simulink model "vdynblksskidpad_final"  (R2026b)
settings: Solver=ode23t  StopTime=inf  RelTol=5e-3
model workspace (MAT data in the model file):
  Eng : object (value not decoded)
  Nmtr = 11.5
  StartupTrim : object (value not decoded)
  SteerLim = 60
  TrackPoints = [-15 -12 -9 -6 -3 5.58745102111e-16 2.81978007367 5.36354042717 7.38228007367 8.67839071119 9.125 8.67839071119 ... (270 elements, 90x3)]
  Trans : object (value not decoded)
  Ts = 0.02
  VEH : object (value not decoded)
values from neighbouring files (symbols this model uses):
  n = size(e.Data,2)    [plot_skidpad_signals.m]
  z = tsMatrix(out.diagWheel.z)    [skidpad_settle_start.m]
symbols that are objects in the model workspace (value not decoded): Eng, StartupTrim, Trans, VEH
undefined symbols (not defined in the file or in its folder): BdyFrm, InertFrm, magnitude
libraries: autolibsharedcoupling x11, simulink x8, sim3dlib x7, autolibshareddiff x5, autolibutils x4, sim3dautolib x3, vehdynlibtirecommon x3, sharedtransform x3, vehdynlibdriver x2, vehdynlibsteering x2, vehdynlibeom x2, vehdynlibviscommon x2
(part 3 of 5)

== system vdynblksskidpad_final/Formula Student Vehicle/Simulink Physics - 7DOF/Powertrain & Driveline/Final Drive/All Wheel Drive ==
  DrvShfTrq : Inport
  Omega : Inport  Port=2
  Demux1 : Demux  Outputs=2
  Demux2 : Demux  Outputs=2
  Demux3 : Demux  Outputs=2
  Limited Slip Differential : autolibshareddiff/Limited Slip Differential  DiffEffModelPopup=Constant  InterpMethod=Linear point-slope  extTamb=off  shaftSwitchMask=To the left of center-line  Ndiff=4  Jd=.1  bd=1e-3  Jw1=.1  bw1=1e-3  Jw2=.1  bw2=1e-3  omegaw1o=0  omegaw2o=0  eta=1  eta_tbl=reshape([0.64 0.76 0.8 0.81 0.83 0.84 0.84 0.56 0.73 0.78 0.8 0.83 0.84 0.84 0.54 0.71 0.77 0.8 0.82 0.84 0.84 0.53 0.71 0.77 0.8 0.83 0.84 0.84 0.51 0.71 0.77 0.8 0.83 0.84 0.85 0.52 0.7 0.77 0.8 0.83 0.84 0.85 0.51 0.71 0.76 0.79 0.83 0.84 0.85 0.5 0.69 0.76 0.79 0.82 0.84 0.85 0.45 0.68 0.75 0.78 0.82 0.84 0.85 0.43 0.67 0.74 0.78 0.81 0.83 0.84 0.38 0.63 0.71 0.75 0.8 0.82 0.83 0.81 0.86 0.88 0.89 0.89 0.89 0.9 0.77 0.85 0.87 0.88 0.89 0.9 0.9 0.72 0.82 0.86 0.87 0.88 0.89 0.9 0.68 0.8 0.84 0.86 0.88 0.89 0.89 0.67 0.8 0.84 0.86 0.88 0.89 0.9 0.67 0.8 0.84 0.86 0.88 0.89 0.9 0.65 0.8 0.84 0.86 0.88 0.89 0.9 0.64 0.79 0.83 0.86 0.88 0.89 0.9 0.63 0.78 0.83 0.86 0.88 0.89 0.9 0.59 0.76 0.82 0.85 0.87 0.89 0.9 0.53 0.73 0.8 0.83 0.86 0.88 0.89], 7, 11, 2)  Trq_bpts=[25, 50, 75, 100, 150, 200, 250]  omega_bpts=[52.4 78.5 105 131 157 183 209 262 314 419 524]  Temp_bpts=[290 358]  Tamb=297.15  couplingType=Pre-loaded ideal clutch  Ndisks=4  Reff=.20  Fc=500  muc=[.16 0.13 0.115 0.11 0.105 0.1025 0.10125]  dw=[0 10 20 40 60 80 100]  Tdw=[-100, -90, -50, -5, 0, 5, 50, 90, 100]  dwT=[-200, -175, -100, - 50, 0, 50, 100, 175, 200]  TTin=[-200 -175 -100 - 50 0 50 100 175 200]  Tin=[-200 -175 -100 - 50 0 50 100 175 200]  tauC=.01  IdealInterpMethod=Linear point-slope  IdealExtrapMethod=Clip  TdwInterpMethod=Linear point-slope  TdwExtrapMethod=Clip  TTinInterpMethod=Linear point-slope  TTinExtrapMethod=Clip  maxAbsSpd=5e3  aMode=2
      settings: LibrarySourceBlock=vdynlib/Powertrain/Drivetrain/Final Drive Unit/Limited Slip Differential
  Open Differential : autolibshareddiff/Open Differential  DiffEffModelPopup=Constant  InterpMethod=Linear point-slope  extTamb=off  shaftSwitchMask=To the left of center-line  Ndiff=4  Jd=.1  bd=1e-3  Jw1=.1  bw1=1e-3  Jw2=.1  bw2=1e-3  omegaw1o=0  omegaw2o=0  eta=1  eta_tbl=reshape([0.64 0.76 0.8 0.81 0.83 0.84 0.84 0.56 0.73 0.78 0.8 0.83 0.84 0.84 0.54 0.71 0.77 0.8 0.82 0.84 0.84 0.53 0.71 0.77 0.8 0.83 0.84 0.84 0.51 0.71 0.77 0.8 0.83 0.84 0.85 0.52 0.7 0.77 0.8 0.83 0.84 0.85 0.51 0.71 0.76 0.79 0.83 0.84 0.85 0.5 0.69 0.76 0.79 0.82 0.84 0.85 0.45 0.68 0.75 0.78 0.82 0.84 0.85 0.43 0.67 0.74 0.78 0.81 0.83 0.84 0.38 0.63 0.71 0.75 0.8 0.82 0.83 0.81 0.86 0.88 0.89 0.89 0.89 0.9 0.77 0.85 0.87 0.88 0.89 0.9 0.9 0.72 0.82 0.86 0.87 0.88 0.89 0.9 0.68 0.8 0.84 0.86 0.88 0.89 0.89 0.67 0.8 0.84 0.86 0.88 0.89 0.9 0.67 0.8 0.84 0.86 0.88 0.89 0.9 0.65 0.8 0.84 0.86 0.88 0.89 0.9 0.64 0.79 0.83 0.86 0.88 0.89 0.9 0.63 0.78 0.83 0.86 0.88 0.89 0.9 0.59 0.76 0.82 0.85 0.87 0.89 0.9 0.53 0.73 0.8 0.83 0.86 0.88 0.89], 7, 11, 2)  Trq_bpts=[25, 50, 75, 100, 150, 200, 250]  omega_bpts=[52.4 78.5 105 131 157 183 209 262 314 419 524]  Temp_bpts=[290 358]  Tamb=297.15  maxAbsSpd=5e3  aMode=2
      settings: LibrarySourceBlock=vdynlib/Powertrain/Drivetrain/Final Drive Unit/Open Differential
  Terminator : Terminator
  Terminator1 : Terminator
  Terminator2 : Terminator
  Torsional Compliance{,1..3} (4 alike) : autolibsharedcoupling/Torsional Compliance  port_config=Simulink  extInfo=off  k=5e3  b=50  theta_o=0  domega_o=0  omega_c=150  blkID=0  aMode=2
      settings: LibrarySourceBlock=vdynlib/Powertrain/Drivetrain/Couplings/Torsional Compliance
  Torsional Compliance4 : autolibsharedcoupling/Torsional Compliance  port_config=Simulink  extInfo=off  k=1e4  b=1e2  theta_o=0  domega_o=0  omega_c=3000  blkID=0  aMode=2
      settings: LibrarySourceBlock=vdynlib/Powertrain/Drivetrain/Couplings/Torsional Compliance
  Torsional Compliance5 : autolibsharedcoupling/Torsional Compliance  port_config=Simulink  extInfo=off  k=1e4  b=1e2  theta_o=0  domega_o=0  omega_c=3000  blkID=0  aMode=2
      settings: LibrarySourceBlock=vdynlib/Powertrain/Drivetrain/Couplings/Torsional Compliance
  Transfer Case : autolibshareddiff/Transfer Case  DiffEffModelPopup=Constant  InterpMethod=Linear point-slope  extTamb=off  TrqSplitRatioMode=off  SpdLockMode=off  shaftSwitchMask=To the left of center-line  Ndiff=1  Jd=.1  bd=1e-3  Jw1=.1  bw1=1e-3  Jw2=.1  bw2=1e-3  omegaw1o=0  omegaw2o=0  eta=1  eta_tbl=reshape([0.64 0.76 0.8 0.81 0.83 0.84 0.84 0.56 0.73 0.78 0.8 0.83 0.84 0.84 0.54 0.71 0.77 0.8 0.82 0.84 0.84 0.53 0.71 0.77 0.8 0.83 0.84 0.84 0.51 0.71 0.77 0.8 0.83 0.84 0.85 0.52 0.7 0.77 0.8 0.83 0.84 0.85 0.51 0.71 0.76 0.79 0.83 0.84 0.85 0.5 0.69 0.76 0.79 0.82 0.84 0.85 0.45 0.68 0.75 0.78 0.82 0.84 0.85 0.43 0.67 0.74 0.78 0.81 0.83 0.84 0.38 0.63 0.71 0.75 0.8 0.82 0.83 0.81 0.86 0.88 0.89 0.89 0.89 0.9 0.77 0.85 0.87 0.88 0.89 0.9 0.9 0.72 0.82 0.86 0.87 0.88 0.89 0.9 0.68 0.8 0.84 0.86 0.88 0.89 0.89 0.67 0.8 0.84 0.86 0.88 0.89 0.9 0.67 0.8 0.84 0.86 0.88 0.89 0.9 0.65 0.8 0.84 0.86 0.88 0.89 0.9 0.64 0.79 0.83 0.86 0.88 0.89 0.9 0.63 0.78 0.83 0.86 0.88 0.89 0.9 0.59 0.76 0.82 0.85 0.87 0.89 0.9 0.53 0.73 0.8 0.83 0.86 0.88 0.89], 7, 11, 2)  Trq_bpts=[25, 50, 75, 100, 150, 200, 250]  omega_bpts=[52.4 78.5 105 131 157 183 209 262 314 419 524]  Temp_bpts=[290 358]  Tamb=297.15  maxAbsSpd=5e3  aMode=2  TrqSplitRatio=0.5  SpdLock=0
      settings: LibrarySourceBlock=vdynlib/Powertrain/Drivetrain/Final Drive Unit/Transfer Case
  Vector Concatenate : Concatenate  NumInputs=4
  AxlTrq : Outport  VectorParamsAs1DForOutWhenUnconnected=off
  AxlSpd : Outport  Port=2  VectorParamsAs1DForOutWhenUnconnected=off
  wires:
  Torsional Compliance2/1 -> Limited Slip Differential/2
  Torsional Compliance3/1 -> Limited Slip Differential/3
  Limited Slip Differential/4 -> Torsional Compliance3/1
  Limited Slip Differential/1 -> Terminator/1
  Demux1/1 -> Torsional Compliance4/2
  Limited Slip Differential/3 -> Torsional Compliance2/1
  Transfer Case/1 -> Terminator1/1
  Transfer Case/2 -> AxlSpd/1
  DrvShfTrq/1 -> Transfer Case/1
  Torsional Compliance3/2 -> Vector Concatenate/4  "T_RR"
  Vector Concatenate/1 -> AxlTrq/1
  Transfer Case/3 -> Torsional Compliance/2
  Transfer Case/4 -> Torsional Compliance1/2
  Torsional Compliance/1 -> Open Differential/1
  Open Differential/2 -> Torsional Compliance/1
  Limited Slip Differential/2 -> Torsional Compliance1/1
  Torsional Compliance1/2 -> Transfer Case/3
  Torsional Compliance/2 -> Transfer Case/2
  Torsional Compliance1/1 -> Limited Slip Differential/1
  Omega/1 -> Demux2/1
  Demux2/1 -> Demux1/1
  Demux2/2 -> Demux3/1
  Demux1/2 -> Torsional Compliance5/2
  Open Differential/3 -> Torsional Compliance4/1
  Open Differential/4 -> Torsional Compliance5/1
  Demux3/1 -> Torsional Compliance2/2
  Demux3/2 -> Torsional Compliance3/2
  Open Differential/1 -> Terminator2/1
  Torsional Compliance4/1 -> Open Differential/2
  Torsional Compliance5/1 -> Open Differential/3
  Torsional Compliance4/2 -> Vector Concatenate/1  "T_FL"
  Torsional Compliance5/2 -> Vector Concatenate/2  "T_FR"
  Torsional Compliance2/2 -> Vector Concatenate/3  "T_RL"

== system vdynblksskidpad_final/Formula Student Vehicle/Simulink Physics - 7DOF/Powertrain & Driveline/Final Drive/Direct ==
  DrvShfTrq : Inport
  Omega : Inport  Port=2
  AxlTrq : Outport  VectorParamsAs1DForOutWhenUnconnected=off
  AxlSpd : Outport  Port=2  VectorParamsAs1DForOutWhenUnconnected=off
  wires:
  Omega/1 -> AxlSpd/1
  DrvShfTrq/1 -> AxlTrq/1

== system vdynblksskidpad_final/Formula Student Vehicle/Simulink Physics - 7DOF/Powertrain & Driveline/Final Drive/Front Wheel Drive ==
  DrvShfTrq : Inport
  Omega : Inport  Port=2
  Demux : Demux  Outputs=[2,2]
  Demux1 : Demux  Outputs=2
  Ground : Ground
  Ground1 : Ground
  Limited Slip Differential : autolibshareddiff/Limited Slip Differential  DiffEffModelPopup=Constant  InterpMethod=Linear point-slope  extTamb=off  shaftSwitchMask=To the left of center-line  Ndiff=Trans.FinalDrive  Jd=.08  bd=1e-3  Jw1=.05  bw1=1e-3  Jw2=.05  bw2=1e-3  omegaw1o=0  omegaw2o=0  eta=1  eta_tbl=reshape([0.64 0.76 0.8 0.81 0.83 0.84 0.84 0.56 0.73 0.78 0.8 0.83 0.84 0.84 0.54 0.71 0.77 0.8 0.82 0.84 0.84 0.53 0.71 0.77 0.8 0.83 0.84 0.84 0.51 0.71 0.77 0.8 0.83 0.84 0.85 0.52 0.7 0.77 0.8 0.83 0.84 0.85 0.51 0.71 0.76 0.79 0.83 0.84 0.85 0.5 0.69 0.76 0.79 0.82 0.84 0.85 0.45 0.68 0.75 0.78 0.82 0.84 0.85 0.43 0.67 0.74 0.78 0.81 0.83 0.84 0.38 0.63 0.71 0.75 0.8 0.82 0.83 0.81 0.86 0.88 0.89 0.89 0.89 0.9 0.77 0.85 0.87 0.88 0.89 0.9 0.9 0.72 0.82 0.86 0.87 0.88 0.89 0.9 0.68 0.8 0.84 0.86 0.88 0.89 0.89 0.67 0.8 0.84 0.86 0.88 0.89 0.9 0.67 0.8 0.84 0.86 0.88 0.89 0.9 0.65 0.8 0.84 0.86 0.88 0.89 0.9 0.64 0.79 0.83 0.86 0.88 0.89 0.9 0.63 0.78 0.83 0.86 0.88 0.89 0.9 0.59 0.76 0.82 0.85 0.87 0.89 0.9 0.53 0.73 0.8 0.83 0.86 0.88 0.89], 7, 11, 2)  Trq_bpts=[25, 50, 75, 100, 150, 200, 250]  omega_bpts=[52.4 78.5 105 131 157 183 209 262 314 419 524]  Temp_bpts=[290 358]  Tamb=297.15  couplingType=Pre-loaded ideal clutch  Ndisks=8  Reff=.08  Fc=1000  muc=[.16 0.13 0.115 0.11 0.105 0.1025 0.10125 .10125]  dw=[0 10 20 40 60 80 100 1000]  Tdw=[-100, -90, -50, -5, 0, 5, 50, 90, 100]  dwT=[-200, -175, -100, - 50, 0, 50, 100, 175, 200]  TTin=[-200 -175 -100 - 50 0 50 100 175 200]  Tin=[-200 -175 -100 - 50 0 50 100 175 200]  tauC=.04  IdealInterpMethod=Linear point-slope  IdealExtrapMethod=Linear  TdwInterpMethod=Flat  TdwExtrapMethod=Clip  TTinInterpMethod=Flat  TTinExtrapMethod=Clip  maxAbsSpd=5e3  aMode=2
      settings: LibrarySourceBlock=vdynlib/Powertrain/Drivetrain/Final Drive Unit/Limited Slip Differential
  Terminator : Terminator
  Terminator1 : Terminator
  Torsional Compliance1 : autolibsharedcoupling/Torsional Compliance  port_config=Simulink  extInfo=off  k=3e5  b=50  theta_o=0  domega_o=0  omega_c=150  blkID=0  aMode=2
      settings: LibrarySourceBlock=vdynlib/Powertrain/Drivetrain/Couplings/Torsional Compliance
  Torsional Compliance2 : autolibsharedcoupling/Torsional Compliance  port_config=Simulink  extInfo=off  k=3e5  b=50  theta_o=0  domega_o=0  omega_c=150  blkID=0  aMode=2
      settings: LibrarySourceBlock=vdynlib/Powertrain/Drivetrain/Couplings/Torsional Compliance
  Vector Concatenate : Concatenate  NumInputs=4
  AxlTrq : Outport  VectorParamsAs1DForOutWhenUnconnected=off
  AxlSpd : Outport  Port=2  VectorParamsAs1DForOutWhenUnconnected=off
  wires:
  Limited Slip Differential/3 -> Torsional Compliance2/1
  Demux1/1 -> Torsional Compliance2/2
  Limited Slip Differential/1 -> Terminator/1
  DrvShfTrq/1 -> Limited Slip Differential/1
  Limited Slip Differential/2 -> AxlSpd/1
  Limited Slip Differential/4 -> Torsional Compliance1/1
  Demux1/2 -> Torsional Compliance1/2
  Demux/1 -> Demux1/1
  Torsional Compliance1/1 -> Limited Slip Differential/3
  Torsional Compliance2/1 -> Limited Slip Differential/2
  Demux/2 -> Terminator1/1
  Ground/1 -> Vector Concatenate/4  "T_RR"
  Torsional Compliance1/2 -> Vector Concatenate/2  "T_FR"
  Ground1/1 -> Vector Concatenate/3  "T_RL"
  Torsional Compliance2/2 -> Vector Concatenate/1  "T_FL"
  Omega/1 -> Demux/1
  Vector Concatenate/1 -> AxlTrq/1

== system vdynblksskidpad_final/Formula Student Vehicle/Simulink Physics - 7DOF/Powertrain & Driveline/Final Drive/Rear Wheel Drive ==
  DrvShfTrq : Inport
  Omega : Inport  Port=2
  Demux : Demux  Outputs=[2,2]
  Demux1 : Demux  Outputs=2
  Ground : Ground
  Ground1 : Ground
  Limited Slip Differential : autolibshareddiff/Limited Slip Differential  DiffEffModelPopup=Constant  InterpMethod=Linear point-slope  extTamb=off  shaftSwitchMask=To the left of center-line  Ndiff=Trans.FinalDrive  Jd=.08  bd=1e-3  Jw1=.01  bw1=1e-3  Jw2=.01  bw2=1e-3  omegaw1o=0  omegaw2o=0  eta=1  eta_tbl=reshape([0.64 0.76 0.8 0.81 0.83 0.84 0.84 0.56 0.73 0.78 0.8 0.83 0.84 0.84 0.54 0.71 0.77 0.8 0.82 0.84 0.84 0.53 0.71 0.77 0.8 0.83 0.84 0.84 0.51 0.71 0.77 0.8 0.83 0.84 0.85 0.52 0.7 0.77 0.8 0.83 0.84 0.85 0.51 0.71 0.76 0.79 0.83 0.84 0.85 0.5 0.69 0.76 0.79 0.82 0.84 0.85 0.45 0.68 0.75 0.78 0.82 0.84 0.85 0.43 0.67 0.74 0.78 0.81 0.83 0.84 0.38 0.63 0.71 0.75 0.8 0.82 0.83 0.81 0.86 0.88 0.89 0.89 0.89 0.9 0.77 0.85 0.87 0.88 0.89 0.9 0.9 0.72 0.82 0.86 0.87 0.88 0.89 0.9 0.68 0.8 0.84 0.86 0.88 0.89 0.89 0.67 0.8 0.84 0.86 0.88 0.89 0.9 0.67 0.8 0.84 0.86 0.88 0.89 0.9 0.65 0.8 0.84 0.86 0.88 0.89 0.9 0.64 0.79 0.83 0.86 0.88 0.89 0.9 0.63 0.78 0.83 0.86 0.88 0.89 0.9 0.59 0.76 0.82 0.85 0.87 0.89 0.9 0.53 0.73 0.8 0.83 0.86 0.88 0.89], 7, 11, 2)  Trq_bpts=[25, 50, 75, 100, 150, 200, 250]  omega_bpts=[52.4 78.5 105 131 157 183 209 262 314 419 524]  Temp_bpts=[290 358]  Tamb=297.15  couplingType=Pre-loaded ideal clutch  Ndisks=4  Reff=.08  Fc=1000  muc=[.16 0.13 0.115 0.11 0.105 0.1025 0.10125 .10125]  dw=[0 10 20 40 60 80 100 1000]  Tdw=[-100, -90, -50, -5, 0, 5, 50, 90, 100]  dwT=[-200, -175, -100, - 50, 0, 50, 100, 175, 200]  TTin=[-200 -175 -100 - 50 0 50 100 175 200]  Tin=[-200 -175 -100 - 50 0 50 100 175 200]  tauC=.04  IdealInterpMethod=Linear point-slope  IdealExtrapMethod=Linear  TdwInterpMethod=Flat  TdwExtrapMethod=Clip  TTinInterpMethod=Flat  TTinExtrapMethod=Clip  maxAbsSpd=5e3  aMode=2
      settings: LibrarySourceBlock=vdynlib/Powertrain/Drivetrain/Final Drive Unit/Limited Slip Differential
  Terminator : Terminator
  Terminator1 : Terminator
  Torsional Compliance : autolibsharedcoupling/Torsional Compliance  port_config=Simulink  extInfo=off  k=5e3  b=50  theta_o=0  domega_o=0  omega_c=600  blkID=0  aMode=2
      settings: LibrarySourceBlock=vdynlib/Powertrain/Drivetrain/Couplings/Torsional Compliance
  Torsional Compliance1 : autolibsharedcoupling/Torsional Compliance  port_config=Simulink  extInfo=off  k=5e3  b=50  theta_o=0  domega_o=0  omega_c=150  blkID=0  aMode=2
      settings: LibrarySourceBlock=vdynlib/Powertrain/Drivetrain/Couplings/Torsional Compliance
  Vector Concatenate : Concatenate  NumInputs=4
  AxlTrq : Outport  VectorParamsAs1DForOutWhenUnconnected=off
  AxlSpd : Outport  Port=2  VectorParamsAs1DForOutWhenUnconnected=off
  wires:
  Torsional Compliance/1 -> Limited Slip Differential/2
  Torsional Compliance1/1 -> Limited Slip Differential/3
  Demux/2 -> Demux1/1
  Demux1/2 -> Torsional Compliance1/2
  Limited Slip Differential/4 -> Torsional Compliance1/1
  Limited Slip Differential/2 -> AxlSpd/1
  DrvShfTrq/1 -> Limited Slip Differential/1
  Limited Slip Differential/1 -> Terminator/1
  Demux1/1 -> Torsional Compliance/2
  Limited Slip Differential/3 -> Torsional Compliance/1
  Demux/1 -> Terminator1/1
  Omega/1 -> Demux/1
  Torsional Compliance1/2 -> Vector Concatenate/4  "T_RR"
  Ground/1 -> Vector Concatenate/2  "T_FR"
  Ground1/1 -> Vector Concatenate/1  "T_FL"
  Torsional Compliance/2 -> Vector Concatenate/3  "T_RL"
  Vector Concatenate/1 -> AxlTrq/1

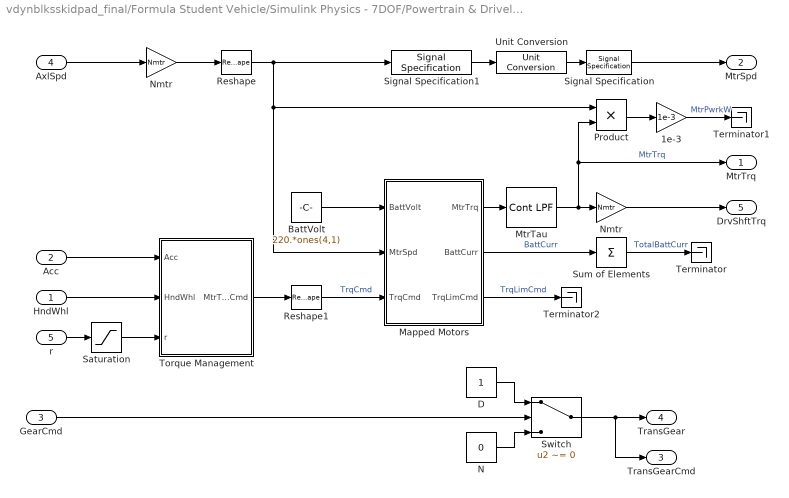
== system vdynblksskidpad_final/Formula Student Vehicle/Simulink Physics - 7DOF/Powertrain & Driveline/Powertrain/4EM Powertrain ==
  HndWhl : Inport
  Acc : Inport  Port=2
  GearCmd : Inport  Port=3
  AxlSpd : Inport  Port=4
  r : Inport  Port=5
  1e-3 : Gain  Gain=1e-3
  BattVolt : Constant  Value=220.*ones(4,1)
  D : Constant
  Mapped Motors : Subsystem
  MtrTau : autolibutils/Cont LPF  wc=200*pi  AbsoluteTolerance=auto  aMode=2
  "N " : Constant  Value=0
  Nmtr : Gain  Gain=Nmtr
  "Nmtr " : Gain  Gain=Nmtr
  Product : Product
  Reshape : Reshape
  Reshape1 : Reshape
  Saturation : Saturate  UpperLimit=500*pi/180  LowerLimit=-500*pi/180  ZeroCross=off
  Signal Specification : SignalSpecification  Unit=rpm
  Signal Specification1 : SignalSpecification  Unit=rad/s
  Sum of Elements : Sum  Inputs=+
  Switch : Switch  Criteria=u2 ~= 0  ZeroCross=off  SaturateOnIntegerOverflow=off  InputSameDT=off
  Terminator : Terminator
  Terminator1 : Terminator
  Terminator2 : Terminator
  Torque Management : MATLAB Function  TreatAsAtomicUnit=on
  Unit Conversion : UnitConversion
  MtrTrq : Outport  VectorParamsAs1DForOutWhenUnconnected=off
  MtrSpd : Outport  Port=2  VectorParamsAs1DForOutWhenUnconnected=off
  TransGearCmd : Outport  Port=3  VectorParamsAs1DForOutWhenUnconnected=off
  TransGear : Outport  Port=4  VectorParamsAs1DForOutWhenUnconnected=off
  DrvShftTrq : Outport  Port=5  VectorParamsAs1DForOutWhenUnconnected=off
  wires:
  Nmtr/1 -> DrvShftTrq/1
  Signal Specification1/1 -> Unit Conversion/1
  Signal Specification/1 -> MtrSpd/1
  "Nmtr "/1 -> Reshape/1
  Unit Conversion/1 -> Signal Specification/1
  Torque Management/1(MtrTrqCmd) -> Reshape1/1
  GearCmd/1 -> Switch/2
  Mapped Motors/1(MtrTrq) -> MtrTau/1
  MtrTau/1 -> Nmtr/1, Product/2, MtrTrq/1  "MtrTrq"
  HndWhl/1 -> Torque Management/2(HndWhl)
  r/1 -> Saturation/1
  Reshape1/1 -> Mapped Motors/3(TrqCmd)  "TrqCmd"
  Switch/1 -> TransGearCmd/1, TransGear/1
  "N "/1 -> Switch/3
  D/1 -> Switch/1
  Saturation/1 -> Torque Management/3(r)
  Acc/1 -> Torque Management/1(Acc)
  AxlSpd/1 -> "Nmtr "/1
  Reshape/1 -> Mapped Motors/2(MtrSpd), Product/1, Signal Specification1/1
  Mapped Motors/2(BattCurr) -> Sum of Elements/1  "BattCurr"
  Sum of Elements/1 -> Terminator/1  "TotalBattCurr"
  Product/1 -> 1e-3/1
  1e-3/1 -> Terminator1/1  "MtrPwrkW"
  BattVolt/1 -> Mapped Motors/1(BattVolt)
  Mapped Motors/3(TrqLimCmd) -> Terminator2/1  "TrqLimCmd"

== system vdynblksskidpad_final/Formula Student Vehicle/Simulink Physics - 7DOF/Powertrain & Driveline/Powertrain/ICE Powertrain ==
  Acc : Inport
  GearCmd : Inport  Port=2
  AxlSpd : Inport  Port=3
  Bus Selector : BusSelector  OutputSignals=Trans.TransGearCmd,Trans.TransGear
  Gain1 : Gain  Gain=100
  Powertrain : autolibutils/Cont LPF  wc=10*pi  AbsoluteTolerance=auto  aMode=2
  Signal Specification : SignalSpecification  Unit=rpm
  Simple Engine : autolibsharedmappedengines/Simple Engine  f_tqmax=Eng.Tbts  f_tqmax_n_bpt=Eng.Nbts  Lhv=4.6E+7  Sg=0.754  BsfcAvg=350  aMode=2
      settings: LibrarySourceBlock=vdynlib/Powertrain/Propulsion/Simple Engine
  Terminator : Terminator
  Transmission : Subsystem  Variant=on  VariantControlMode=label  LabelModeActiveChoice=0
  MtrTrq : Outport  VectorParamsAs1DForOutWhenUnconnected=off
  MtrSpd : Outport  Port=2  VectorParamsAs1DForOutWhenUnconnected=off
  TransGearCmd : Outport  Port=3  VectorParamsAs1DForOutWhenUnconnected=off
  TransGear : Outport  Port=4  VectorParamsAs1DForOutWhenUnconnected=off
  DrvShftTrq : Outport  Port=5  VectorParamsAs1DForOutWhenUnconnected=off
  wires:
  Acc/1 -> Gain1/1
  Signal Specification/1 -> Simple Engine/2, MtrSpd/1
  Simple Engine/2 -> Powertrain/1
  Gain1/1 -> Simple Engine/1
  Transmission/1(EngSpd) -> Signal Specification/1
  Simple Engine/1 -> Terminator/1
  Transmission/2(Info) -> Bus Selector/1
  Bus Selector/1 -> TransGearCmd/1  "<TransGearCmd>"
  Bus Selector/2 -> TransGear/1  "<TransGear>"
  GearCmd/1 -> Transmission/2(GearCmd)
  Powertrain/1 -> Transmission/1(EngTrq), MtrTrq/1
  Transmission/3(DrvShfTrq) -> DrvShftTrq/1
  AxlSpd/1 -> Transmission/3(PropShftSpd)

== system vdynblksskidpad_final/Visualization/3D Visualization/Enabled/3D Visualization/Disabled ==

== system vdynblksskidpad_final/Visualization/3D Visualization/Enabled/3D Visualization/Ground Following ==
  VehFdbk : Inport
  Annotations : Subsystem  Variant=on  VariantControl=Annotations
  Bus Selector3 : BusSelector  OutputSignals=VehFdbk.InertFrm.Cg.Disp.X,VehFdbk.InertFrm.Cg.Disp.Y,VehFdbk.InertFrm.Cg.Ang.psi,Driver.Light controls
  Path : Subsystem  Variant=on  VariantControl=Choice
  Simulation 3D Scene Configuration : sim3dlib/Simulation 3D Scene Configuration  Priority=0  ProjectFormat=Default Scenes  SceneDesc=Open surface  ProjectName=/mathworks/devel/bat/filer/batfs2566-0/Bdoc25b.3168145/build/runnable/matlab/toolbox/shared/sim3d_projects/automotive_project_linux/UE/LinuxNoEditor/VehicleSimulation.sh  ScenePath=/Game/Maps/HwStrght  EnableOpenDRIVE=off  vehTagList={'Custom';'GamePhysVehPath';'GrndVehPath';'Scene Origin';'Sim3dActor1';'SimulinkPhysVehPath';'SimulinkVehicle1';'SimulinkVehicle2';'SimulinkVehicle3'}  vehTag=SimulinkVehicle3  AttachedCameraRelativeTranslation=[0 0 0]  FreeCameraDefaultInitialTranslation=[-6, 0, 2]  AttachedCameraRelativeRotation=[0 0 0]  FreeCameraDefaultInitialRotation=[0, -15, 0]  ViewpointName=Custom  FreeCameraInitialTranslation=[0 0 0]  ViewpointTranslation=[0 0 0]  FreeCameraInitialRotation=[0 0 0]  ViewpointRotation=[0 0 0]  OpVisEn=off  Ts=Ts  EnableWindow=on  EnableRemoteAccess=off  EnableWeather=off  SunAzimuth=90  SunAltitude=40.0  EnableGeospatialSun=off  Latitude=0  Longitude=0  Date=2023-01-01  Time=10:30:00  GeoTimeZone=-5.0  SunDaylightSaving=off  wind=1  clouds=10  EnableVolumetricClouds=off  CloudCoverage=0  CloudAltitude=6  fog=0  rain=0  RaindropsEffect=off  SnowDensity=0  EnableGeospatial=off  TilesetSource=Earth terrain  UseTrueOrigin=off  OriginHeight=200  OriginLatitude=40.744652  OriginLongitude=-73.988864  MapStyle=Aerial  AdditionalAssetIDs=[]  UseAdvancedSunSky=off  SolarTime=11  TimeZone=-5  Day=21  Month=9  Year=2022  UseDaylightSavingTime=on  DSTStartDay=10  DSTStartMonth=3  DSTEndDay=3  DSTEndMonth=11  DSTSwitchHour=2  sensorTag=MainCamera1  sensorId=1  sensorName=MainCamera1  mountLoc=Origin  offsetFlag=off  tmountOffset=[0, 0, 0]  rmountOffset=[0, 0, 0]  HorizontalResolution=1280  VerticalResolution=720  HorizontalFOV=60  mountPoint=[0 0 0]  mountOrientation=[0 0 0]  aMode=2  ID=1  GeoTrigger=Inactive  ViewNameList={'Custom'}  ViewTranslationList={'[0 0 0]'}  ViewRotationList={'[0 0 0]'}
      settings: LibrarySourceBlock=vdynlib/Vehicle Scenarios/Sim3D/Sim3D Core/Simulation 3D Scene Configuration
  Simulation 3D Vehicle with Ground Following : sim3dautolib/Simulation 3D Vehicle with Ground Following VDBS  Priority=-1  PassVehMesh=Hatchback  MeshPath=/MathWorksSimulation/Vehicles/Muscle/Meshes/SK_MuscleCar.SK_MuscleCar  TrackWidth=1.9  WheelBase=3  WheelRadius=0.35  VehColor=Red  CoordinateSystem=SAE  InitialPos=[ VEH.InitialLongPosition, VEH.InitialLatPosition, VEH.InitialVertPosition ]  InitialRot=[VEH.InitialRollAngle VEH.InitialPitchAngle VEH.InitialYawAngle]  ActorName=SimulinkVehicle3  VehLightsControl=on  HeadlightColor=[ 1, 1, 1 ]  HighBeamIntensity=100000  LowBeamIntensity=60000  HighBeamConeAngle=1.22  LowBeamConeAngle=1.22  LeftHeadlightOrientation=[ 0, 0 ]  RightHeadlightOrientation=[ 0, 0 ]  BrakelightIntensity=200  ReverselightIntensity=500  SignallightIntensity=500  SignallightPeriod=1  SignalPulseWidth=50  SampleTime=Ts  ActorType=SimulinkVehicle  ID=3  aMode=2  ActorTag=SimulinkVehicle3  CoordinateScheme=SAE
      settings: LibrarySourceBlock=vehdynlibsim3d/Simulation 3D Vehicle with Ground Following
  wires:
  Bus Selector3/1 -> Simulation 3D Vehicle with Ground Following/1  "<X>"
  VehFdbk/1 -> Path/1(VehFdbk), Annotations/1(VehFdbk), Bus Selector3/1
  Bus Selector3/2 -> Simulation 3D Vehicle with Ground Following/2  "<Y>"
  Bus Selector3/4 -> Simulation 3D Vehicle with Ground Following/4  "<Light controls>"
  Bus Selector3/3 -> Simulation 3D Vehicle with Ground Following/3  "<psi>"

== system vdynblksskidpad_final/Visualization/3D Visualization/Enabled/3D Visualization/Physical Vehicle ==
  VehFdbk : Inport
  Annotations : Subsystem  Variant=on  VariantControl=Annotations
  Path : Subsystem  Variant=on  VariantControl=Choice
  Simulation 3D Scene Configuration : sim3dlib/Simulation 3D Scene Configuration  Priority=0  ProjectFormat=Default Scenes  SceneDesc=Open surface  ProjectName=/mathworks/devel/bat/filer/batfs2566-0/Bdoc25b.3168145/build/runnable/matlab/toolbox/shared/sim3d_projects/automotive_project_linux/UE/LinuxNoEditor/VehicleSimulation.sh  ScenePath=/Game/Maps/HwStrght  UEProjPath=L:\Bsim3d\scm\automotive_project_UE4\main\src\main\AutoVrtlEnv\AutoVrtlEnv.uproject  EnableOpenDRIVE=off  vehTagList={'Custom';'GamePhysVehPath';'GrndVehPath';'Scene Origin';'Sim3dActor1';'SimulinkPhysVehPath';'SimulinkVehicle1';'SimulinkVehicle2';'SimulinkVehicle3'}  vehTag=SimulinkVehicle2  AttachedCameraRelativeTranslation=[0 0 0]  FreeCameraDefaultInitialTranslation=[-6, 0, 2]  AttachedCameraRelativeRotation=[0 0 0]  FreeCameraDefaultInitialRotation=[0, -15, 0]  ViewpointName=Custom  FreeCameraInitialTranslation=[0 0 0]  ViewpointTranslation=[0 0 0]  FreeCameraInitialRotation=[0 0 0]  ViewpointRotation=[0 0 0]  OpVisEn=off  Ts=Ts  EnableWindow=on  EnableRemoteAccess=off  EnableWeather=off  SunAzimuth=90  SunAltitude=40.0  EnableGeospatialSun=off  Latitude=0  Longitude=0  Date=2023-01-01  Time=10:30:00  GeoTimeZone=-5.0  SunDaylightSaving=off  wind=1  clouds=10  EnableVolumetricClouds=off  CloudCoverage=0  CloudAltitude=6  fog=0  rain=0  RaindropsEffect=off  SnowDensity=0  EnableGeospatial=off  TilesetSource=Earth terrain  UseTrueOrigin=off  OriginHeight=200  OriginLatitude=40.744652  OriginLongitude=-73.988864  MapStyle=Aerial  AdditionalAssetIDs=[]  UseAdvancedSunSky=off  SolarTime=11  TimeZone=-5  Day=21  Month=9  Year=2022  UseDaylightSavingTime=on  DSTStartDay=10  DSTStartMonth=3  DSTEndDay=3  DSTEndMonth=11  DSTSwitchHour=2  sensorTag=MainCamera2  sensorId=2  sensorName=MainCamera2  mountLoc=Origin  offsetFlag=off  tmountOffset=[0, 0, 0]  rmountOffset=[0, 0, 0]  HorizontalResolution=1280  VerticalResolution=720  HorizontalFOV=60  mountPoint=[0 0 0]  mountOrientation=[0 0 0]  aMode=2  ID=2  GeoTrigger=Inactive  ViewNameList={'Custom'}  ViewTranslationList={'[0 0 0]'}  ViewRotationList={'[0 0 0]'}
      settings: LibrarySourceBlock=vdynlib/Vehicle Scenarios/Sim3D/Sim3D Core/Simulation 3D Scene Configuration
  wires:
  VehFdbk/1 -> Path/1(VehFdbk), Annotations/1(VehFdbk)

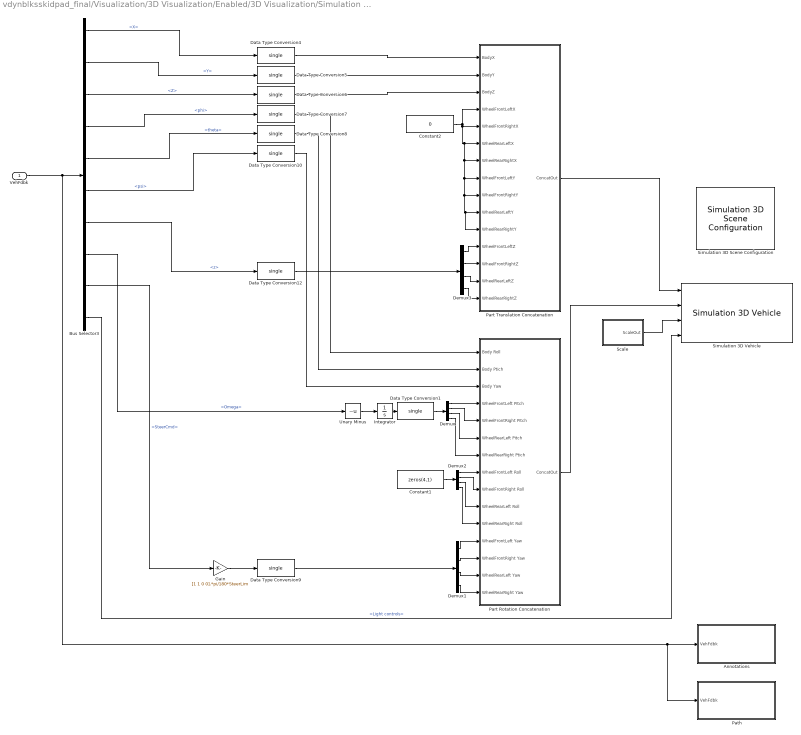
== system vdynblksskidpad_final/Visualization/3D Visualization/Enabled/3D Visualization/Simulation 3D Vehicle ==
  VehFdbk : Inport
  Annotations : Subsystem  Variant=on  VariantControl=Annotations
  Bus Selector3 : BusSelector  OutputSignals=VehFdbk.InertFrm.Cg.Disp.X,VehFdbk.InertFrm.Cg.Disp.Y,VehFdbk.InertFrm.Cg.Disp.Z,VehFdbk.InertFrm.Cg.Ang.phi,VehFdbk.InertFrm.Cg.Ang.theta,VehFdbk.InertFrm.Cg.Ang.psi,VehFdbk.Wheels.z,VehFdbk.Wheels.Omega,Driver.SteerCmd,Driver.Light controls
  Constant1 : Constant  Value=zeros(4,1)  OutDataTypeStr=single
  Constant2 : Constant  Value=0  OutDataTypeStr=single
  Data Type Conversion{1,4..10,12} (9 alike) : DataTypeConversion  OutDataTypeStr=single  SaturateOnIntegerOverflow=off  RndMeth=Floor
  Demux{,1..3} (4 alike) : Demux
  Gain : Gain  Gain=[1 1 0 0].*pi/180*SteerLim
  Integrator : Integrator  WrapState=on  WrappedStateUpperValue=2*pi  WrappedStateLowerValue=0  ZeroCross=off
  Part Rotation Concatenation : Subsystem
  Part Translation Concatenation : Subsystem
  Path : Subsystem  Variant=on  VariantControl=Choice
  Scale : Subsystem
  Simulation 3D Scene Configuration : sim3dlib/Simulation 3D Scene Configuration  Priority=0  ProjectFormat=Default Scenes  SceneDesc=Open surface  ProjectName=/mathworks/devel/bat/filer/batfs2566-0/Bdoc25b.3168145/build/runnable/matlab/toolbox/shared/sim3d_projects/automotive_project_linux/UE/LinuxNoEditor/VehicleSimulation.sh  ScenePath=/Game/Maps/BlackLake  EnableOpenDRIVE=off  vehTagList={'Custom';'GamePhysVehPath';'GrndVehPath';'Scene Origin';'Sim3dActor1';'SimulinkPhysVehPath';'SimulinkVehicle1';'SimulinkVehicle2';'SimulinkVehicle3'}  vehTag=SimulinkVehicle1  AttachedCameraRelativeTranslation=[0 0 0]  FreeCameraDefaultInitialTranslation=[-6, 0, 2]  AttachedCameraRelativeRotation=[0 0 0]  FreeCameraDefaultInitialRotation=[0, -15, 0]  ViewpointName=Custom  FreeCameraInitialTranslation=[0 0 0]  ViewpointTranslation=[0 0 0]  FreeCameraInitialRotation=[0 0 0]  ViewpointRotation=[0 0 0]  OpVisEn=off  Ts=Ts  EnableWindow=on  EnableRemoteAccess=off  EnableWeather=off  SunAzimuth=90  SunAltitude=40.0  EnableGeospatialSun=off  Latitude=0  Longitude=0  Date=2023-01-01  Time=10:30:00  GeoTimeZone=-5.0  SunDaylightSaving=off  wind=1  clouds=10  EnableVolumetricClouds=off  CloudCoverage=0  CloudAltitude=6  fog=0  rain=0  RaindropsEffect=off  SnowDensity=0  EnableGeospatial=off  TilesetSource=Earth terrain  UseTrueOrigin=off  OriginHeight=200  OriginLatitude=40.744652  OriginLongitude=-73.988864  MapStyle=Aerial  AdditionalAssetIDs=[]  UseAdvancedSunSky=off  SolarTime=11  TimeZone=-5  Day=21  Month=9  Year=2022  UseDaylightSavingTime=on  DSTStartDay=10  DSTStartMonth=3  DSTEndDay=3  DSTEndMonth=11  DSTSwitchHour=2  sensorTag=MainCamera3  sensorId=3  sensorName=MainCamera3  mountLoc=Origin  offsetFlag=off  tmountOffset=[0, 0, 0]  rmountOffset=[0, 0, 0]  HorizontalResolution=1280  VerticalResolution=720  HorizontalFOV=60  mountPoint=[0 0 0]  mountOrientation=[0 0 0]  aMode=2  ID=3  GeoTrigger=Inactive  ViewNameList={'Custom'}  ViewTranslationList={'[0 0 0]'}  ViewRotationList={'[0 0 0]'}
      settings: LibrarySourceBlock=vdynlib/Vehicle Scenarios/Sim3D/Sim3D Core/Simulation 3D Scene Configuration
  Simulation 3D Vehicle : sim3dautolib/Simulation 3D Vehicle  Priority=-1  PassVehMesh=Formula student vehicle  MeshPath=/MathWorksSimulation/Vehicles/Muscle/Meshes/SK_MuscleCar.SK_MuscleCar  VehColor=Red  ActorName=SimulinkVehicle1  VehLightsControl=on  HeadlightColor=[ 1, 1, 1 ]  HighBeamIntensity=100000  LowBeamIntensity=60000  HighBeamConeAngle=1.22  LowBeamConeAngle=1.22  LeftHeadlightOrientation=[ 0, 0 ]  RightHeadlightOrientation=[ 0, 0 ]  BrakelightIntensity=500  ReverselightIntensity=500  SignallightIntensity=500  SignallightPeriod=1  SignalPulseWidth=50  Translation=[ VEH.InitialLongPosition, VEH.InitialLatPosition, VEH.InitialVertPosition *0; zeros(4,3)]  Rotation=[VEH.InitialRollAngle VEH.InitialPitchAngle VEH.InitialYawAngle; zeros( 4, 3 )]  Scale=ones( 5, 3 )  SampleTime=Ts  ActorType=SimulinkVehicle  ID=1  aMode=2  ActorTag=SimulinkVehicle1
      settings: LibrarySourceBlock=vdynlib/Vehicle Scenarios/Sim3D/Sim3D Vehicle/Components/Simulation 3D Vehicle
  Unary Minus : UnaryMinus
  wires:
  Bus Selector3/6 -> Data Type Conversion10/1  "<psi>"
  Bus Selector3/10 -> Simulation 3D Vehicle/4  "<Light controls>"
  Bus Selector3/2 -> Data Type Conversion5/1  "<Y>"
  VehFdbk/1 -> Path/1(VehFdbk), Annotations/1(VehFdbk), Bus Selector3/1
  Bus Selector3/1 -> Data Type Conversion4/1  "<X>"
  Data Type Conversion10/1 -> Part Rotation Concatenation/3(Body Yaw)
  Data Type Conversion5/1 -> Part Translation Concatenation/2(BodyY)
  Constant2/1 -> Part Translation Concatenation/5(WheelFrontRightX), Part Translation Concatenation/6(WheelRearLeftX), Part Translation Concatenation/7(WheelRearRightX), Part Translation Concatenation/8(WheelFrontLeftY), Part Translation Concatenation/9(WheelFrontRightY), Part Translation Concatenation/10(WheelRearLeftY), Part Translation Concatenation/11(WheelRearRightY), Part Translation Concatenation/4(WheelFrontLeftX)
  Data Type Conversion8/1 -> Part Rotation Concatenation/2(Body Ptich)
  Demux2/2 -> Part Rotation Concatenation/9(WheelFrontRight Roll)
  Demux1/3 -> Part Rotation Concatenation/14(WheelRearLeft Yaw)
  Demux/3 -> Part Rotation Concatenation/6(WheelRearLeft Pitch)
  Data Type Conversion9/1 -> Demux1/1
  Demux1/2 -> Part Rotation Concatenation/13(WheelFrontRight Yaw)
  Demux/2 -> Part Rotation Concatenation/5(WheelFrontRight Pitch)
  Demux2/3 -> Part Rotation Concatenation/10(WheelRearLeft Roll)
  Bus Selector3/5 -> Data Type Conversion8/1  "<theta>"
  Data Type Conversion7/1 -> Part Rotation Concatenation/1(Body Roll)
  Demux3/2 -> Part Translation Concatenation/13(WheelFrontRightZ)
  Data Type Conversion4/1 -> Part Translation Concatenation/1(BodyX)
  Integrator/1 -> Data Type Conversion1/1
  Demux2/1 -> Part Rotation Concatenation/8(WheelFrontLeft Roll)
  Demux1/4 -> Part Rotation Concatenation/15(WheelRearRight Yaw)
  Demux3/4 -> Part Translation Concatenation/15(WheelRearRightZ)
  Bus Selector3/4 -> Data Type Conversion7/1  "<phi>"
  Bus Selector3/7 -> Data Type Conversion12/1  "<z>"
  Bus Selector3/8 -> Unary Minus/1  "<Omega>"
  Data Type Conversion1/1 -> Demux/1
  Constant1/1 -> Demux2/1
  Demux3/3 -> Part Translation Concatenation/14(WheelRearLeftZ)
  Part Rotation Concatenation/1(ConcatOut) -> Simulation 3D Vehicle/2
  Demux3/1 -> Part Translation Concatenation/12(WheelFrontLeftZ)
  Part Translation Concatenation/1(ConcatOut) -> Simulation 3D Vehicle/1
  Demux/1 -> Part Rotation Concatenation/4(WheelFrontLeft Pitch)
  Demux1/1 -> Part Rotation Concatenation/12(WheelFrontLeft Yaw)
  Data Type Conversion6/1 -> Part Translation Concatenation/3(BodyZ)
  Unary Minus/1 -> Integrator/1
  Demux/4 -> Part Rotation Concatenation/7(WheelRearRight Ptich)
  Demux2/4 -> Part Rotation Concatenation/11(WheelRearRight Roll)
  Data Type Conversion12/1 -> Demux3/1
  Scale/1(ScaleOut) -> Simulation 3D Vehicle/3
  Bus Selector3/3 -> Data Type Conversion6/1  "<Z>"
  Bus Selector3/9 -> Gain/1  "<SteerCmd>"
  Gain/1 -> Data Type Conversion9/1

== system vdynblksskidpad_final/Visualization/3D Visualization/Enabled/Cones/Disabled ==

== system vdynblksskidpad_final/Visualization/3D Visualization/Enabled/Cones/Enabled ==
  Simulation 3D Actor : sim3dlib/Simulation 3D Actor  ActorName=Sim3dActor1  ParentName=Scene Origin  Operation=Create at setup  InitScriptText=|  SampleTime=Ts  Translation=single([0 0 0])  Rotation=single([0 0 0])  Scale=single([1 1 1])  aMode=5  ActorTag=Sim3dActor1  ActorType=Sim3dActor  ID=1
      | entryWidth =3.453;
      | conesZ0 = 0;
      | entryConesLoc = [entryWidth/2 -12;...
      |                  -entryWidth/2 -12;...
      |                  -entryWidth/2 -10;...
      |                  entryWidth/2 -10];
      | entryConesLoc= fliplr(entryConesLoc); % account for game engine coords
      | rightInnerRingLoc = [entryWidth/2 0;...%1
      |                   4.58/2 -2.834;...%2
      |                   7.787/2 -5.231;...%3
      |                   12.588/2 -6.835;...%4
      |                   18.25/2 -7.398;...%5
      |                   23.912/2 -6.835;...%6
      |                   28.713/2 -5.231;...%7
      |                   31.92/2 -2.834;...%8
      |                   33.047/2 0;...%9
      |                   31.92/2 2.834;...%10
      |                   28.713/2 5.231;...%11
      |                   23.912/2 6.835;...%12
      |                   18.25/2 7.398;...%13
      |                   12.588/2 6.835;...%14
      |                   7.787/2 5.231;...%15
      |                   4.58/2 2.834;...%16    
      |                   ];
      | rightInnerRingLoc = fliplr(rightInnerRingLoc);
      | leftInnerRingLoc = rightInnerRingLoc.*[1 -1];
      | rightOutterRingLoc = [entryWidth/2 7.939;...% right side entry to exit zone
      |                       9.945/2 10.026;...
      |                       18.25/2 10.852;...
      |                       26.555/2 10.026;...
      |                       33.596/2 7.673;...
      |                       38.301/2 4.153;...
      |                       39.953/2 0;...
      |                       38.301/2 -4.153;...
      |                       33.596/2 -7.673;...
      |                       26.555/2 -10.026;...
      |                       18.25/2 -10.852;...
      |                       9.945/2 -10.026;...                      
      |                       entryWidth/2 -7.939;...% right side after entry zone                      
      |                       ];
      | rightOutterRingLoc = fliplr(rightOutterRingLoc);
      | leftOutterRingLoc = rightOutterRingLoc.*[1 -1];
      | 
      | exitConesLoc = [entryWidth/2 16;...
      |                  -entryWidth/2 16;...
      |                  entryWidth/2-1 16;...
      |                  -entryWidth/2+1 16;...
      |                  -entryWidth/2 14;...
      |                  entryWidth/2 14;...
      |                  -entryWidth/2 12;...
      |                  entryWidth/2 12;...
      |                  -entryWidth/2 10;...
      |                  entryWidth/2 10];
      | exitConesLoc= fliplr(exitConesLoc); % account for game engine coords
      | 
      | timeConesLoc = fliplr([entryWidth/2 .5;...
      |                  -entryWidth/2 .5;...
      |                  entryWidth/2 -.5;...
      |                  -entryWidth/2 -.5]);
      | 
      | blueCones = [rightOutterRingLoc; leftInnerRingLoc];
      | yellowCones = [rightInnerRingLoc; leftOutterRingLoc];
      | smallOrangeCones = [entryConesLoc; exitConesLoc];
      | largeOrangeCones = timeConesLoc;
      | 
      | skidSurface = sim3d.Actor('ActorName','BaseSurface');
      | skidSurface.createShape('box',[45,45,+0.03]);
      | skidSurface.Color = [68 68 71]./100;
      | skidSurface.Translation = [0 0 0]; 
      | skidSurface.Texture = fullfile(pwd,"vdynskidpad.png"); 
      | skidSurface.TextureTransform.Scale = [1 1];
      | skidSurface.TextureTransform.Angle = 0;
      | skidSurface.Shininess = 0;
      | skidSurface.Transparency = 0;
      | skidSurface.TextureMapping.Blend = 1;
      | skidSurface.TextureMapping.Roughness = .8;
      | World.add(skidSurface,Actor);
      | 
      | nCones = length(largeOrangeCones);
      | for coneNum = 1:nCones    
      |     coneName = "LCone_" + num2str(coneNum);
      |     conLoc = [largeOrangeCones(coneNum,:) conesZ0];
      |     cone = sim3d.Actor('ActorName',coneName,'Mesh','/Game/Environment/Industrial/Props/Cone/Mesh/SM_Cone.SM_Cone',...
      |         'Mobility', sim3d.utils.MobilityTypes.Movable,...
      |         'SimulatePhysics', true,...
      |         'Translation',conLoc,...
      |         'EnableGravity', true);    
      |     %cone.Shadows = true;
      |     World.add(cone,Actor);
      | end
      | 
      | %smallCones = [blueCones; yellowCones; smallOrangeCones]; 
      | 
      | 
      | for coneNum = 1:length(blueCones)    
      |     coneName = "bCone_" + num2str(coneNum);
      |     conLoc = [blueCones(coneNum,:) conesZ0];
      |     cone = sim3d.Actor('ActorName',coneName,'Mesh','/Game/Environment/Industrial/Props/Cone/Mesh/SM_Cone_Blue.SM_Cone_Blue',...
      |         'Mobility', sim3d.utils.MobilityTypes.Movable,...
      |         'SimulatePhysics', true,...
      |         'Translation',conLoc,...
      |         'EnableGravity', true,...
      |         'Scale',ones(1,3).*325/500);    
      |     %cone.Color= [102 140 204]./255;
      |     World.add(cone,Actor);
      | end
      | for coneNum = 1:length(yellowCones)    
      |     coneName = "yCone_" + num2str(coneNum);
      |     conLoc = [yellowCones(coneNum,:) conesZ0];
      |     cone = sim3d.Actor('ActorName',coneName,'Mesh','/Game/Environment/Industrial/Props/Cone/Mesh/SM_Cone_Yellow.SM_Cone_Yellow',...
      |         'Mobility', sim3d.utils.MobilityTypes.Movable,...
      |         'SimulatePhysics', true,...
      |         'Translation',conLoc,...
      |         'EnableGravity', true,...
      |         'Scale',ones(1,3).*325/500);    
      |     %cone.Color= [102 140 204]./255;
      |     World.add(cone,Actor);
      | end
      | for coneNum = 1:length(smallOrangeCones)    
      |     coneName = "sCone_" + num2str(coneNum);
      |     conLoc = [smallOrangeCones(coneNum,:) conesZ0];
      |     cone = sim3d.Actor('ActorName',coneName,'Mesh','/Game/Environment/Industrial/Props/Cone/Mesh/SM_Cone.SM_Cone',...
      |         'Mobility', sim3d.utils.MobilityTypes.Movable,...
      |         'SimulatePhysics', true,...
      |         'Translation',conLoc,...
      |         'EnableGravity', true,...
      |         'Scale',ones(1,3).*325/500);    
      |     %cone.Color= [102 140 204]./255;
      |     World.add(cone,Actor);
      | end
      settings: LibrarySourceBlock=sl3dlib/Simulation 3D/Simulation 3D Actor
  Terminator : Terminator
  wires:
  Simulation 3D Actor/1 -> Terminator/1

== system vdynblksskidpad_final/Formula Student Vehicle/Simulink Physics - 7DOF/Powertrain & Driveline/Brakes and Wheels/Tire2Veh/Wheel Angles ==
  Front : Inport
  Camber : Inport  Port=2
  Constant : Constant  Value=zeros(4,1)
  MATLAB Function : Gain  Gain=[0 0 1]  Multiplication=Matrix(K*u)
  Reshape : Reshape  OutputDimensionality=Row vector (2-D)
  Reshape1 : Reshape  OutputDimensionality=Row vector (2-D)
  Reshape2 : Reshape  OutputDimensionality=Row vector (2-D)
  Vector Concatenate3 : Concatenate  NumInputs=3  Mode=Multidimensional array
  Vehicle : Outport  VectorParamsAs1DForOutWhenUnconnected=off
  wires:
  Reshape/1 -> Vector Concatenate3/3
  Reshape2/1 -> Vector Concatenate3/2
  Vector Concatenate3/1 -> Vehicle/1
  Reshape1/1 -> Vector Concatenate3/1
  Camber/1 -> Reshape1/1
  Constant/1 -> Reshape2/1
  Front/1 -> MATLAB Function/1
  MATLAB Function/1 -> Reshape/1

== system vdynblksskidpad_final/Formula Student Vehicle/Simulink Physics - 7DOF/Powertrain & Driveline/Brakes and Wheels/Tire2Veh/Wheel to Body Transform ==
  Forces : Inport  PortDimensions=[3,1]  Partition=on  PartitionDimension=2  PartitionWidth=1  PartitionOffset=0
  WheelAngles : Inport  Port=2  Partition=on  PartitionDimension=2  PartitionWidth=1  PartitionOffset=0
  Constant : Constant  Value=[pi;0;0]
  Demux1 : Demux  Outputs=3
  Divide1 : Product  Inputs=***  Multiplication=Matrix(*)
  For Each : ForEach  DisableCoverage=on
  Rotation Angles to Direction Cosine Matrix : sharedtransform/Rotation Angles to Direction Cosine Matrix  rotationOrder=ZYX  aMode=2
  Rotation Angles to Direction Cosine Matrix1 : sharedtransform/Rotation Angles to Direction Cosine Matrix  rotationOrder=ZYX  aMode=2
  Selector : Selector  InputPortWidth=3  IndexOptions=Index vector (dialog)  Indices=[3 2 1]  OutputSizes=1  RuntimeRangeChecks=off
  Selector1 : Selector  InputPortWidth=3  IndexOptions=Index vector (dialog)  Indices=[3 2 1]  OutputSizes=1  RuntimeRangeChecks=off
  Transpose : Math  Operator=transpose
  Fx : Outport  ConcatenationDimension=1  VectorParamsAs1DForOutWhenUnconnected=off
  Fy : Outport  Port=2  ConcatenationDimension=1  VectorParamsAs1DForOutWhenUnconnected=off
  Fz : Outport  Port=3  ConcatenationDimension=1  VectorParamsAs1DForOutWhenUnconnected=off
  wires:
  Demux1/1 -> Fx/1
  Demux1/2 -> Fy/1
  Demux1/3 -> Fz/1
  Rotation Angles to Direction Cosine Matrix/1 -> Transpose/1
  Forces/1 -> Divide1/3
  WheelAngles/1 -> Selector/1
  Selector/1 -> Rotation Angles to Direction Cosine Matrix/1
  Rotation Angles to Direction Cosine Matrix1/1 -> Divide1/2
  Divide1/1 -> Demux1/1
  Selector1/1 -> Rotation Angles to Direction Cosine Matrix1/1
  Constant/1 -> Selector1/1
  Transpose/1 -> Divide1/1

== system vdynblksskidpad_final/Formula Student Vehicle/Simulink Physics - 7DOF/Powertrain & Driveline/Brakes and Wheels/Veh2Tire/Wheel to Body Transform ==
  VelVeh : Inport  Partition=on  PartitionDimension=2  PartitionWidth=1  PartitionOffset=0
  WhlAng : Inport  Port=2  Partition=on  PartitionDimension=2  PartitionWidth=1  PartitionOffset=0
  Demux1 : Demux  Outputs=3
  Divide1 : Product  Inputs=**  Multiplication=Matrix(*)
  For Each : ForEach  DisableCoverage=on
  Rotation Angles to Direction Cosine Matrix : sharedtransform/Rotation Angles to Direction Cosine Matrix  rotationOrder=ZYX  aMode=2
  Selector : Selector  InputPortWidth=3  IndexOptions=Index vector (dialog)  Indices=[3 2 1]  OutputSizes=1  RuntimeRangeChecks=off
  xdotWheel : Outport  ConcatenationDimension=1  VectorParamsAs1DForOutWhenUnconnected=off
  ydotWheel : Outport  Port=2  ConcatenationDimension=1  VectorParamsAs1DForOutWhenUnconnected=off
  zdotWheel : Outport  Port=3  ConcatenationDimension=1  VectorParamsAs1DForOutWhenUnconnected=off
  wires:
  Divide1/1 -> Demux1/1
  Demux1/1 -> xdotWheel/1
  Demux1/2 -> ydotWheel/1
  Demux1/3 -> zdotWheel/1
  Rotation Angles to Direction Cosine Matrix/1 -> Divide1/1
  VelVeh/1 -> Divide1/2
  WhlAng/1 -> Selector/1
  Selector/1 -> Rotation Angles to Direction Cosine Matrix/1
